simulink model "stsmc"  (R2026a)
settings: Solver=FixedStepDiscrete  FixedStep=0.001
undefined symbols (not defined in the file): DiscIntNeverNeededParam
libraries: discretizing x2
settings Model: SILPILModeSetting=veronly  Creator=HomePC  LastModifiedBy=HomePC
settings RTWCC: SystemTargetFile=ert.tlc  GenCodeOnly=on  TemplateMakefile=RTW.MSVCBuild  Toolchain=ESP32  BuildConfiguration=Faster Runs  Description=Create Visual C/C++ Solution File for Embedded Coder
settings ERTTargetCC: DynamicArrayContainerType=coder::array  GenerateSampleERTMain=on  SupportComplex=off

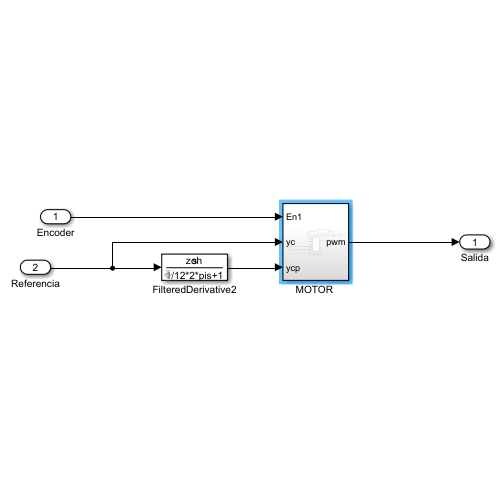
[thumbnail: Simulink's stored preview of the top-level diagram]
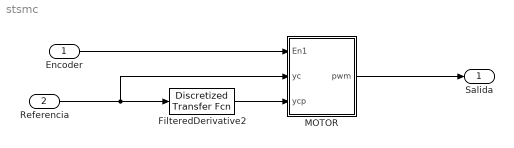
== system stsmc ==
  Encoder : Inport
  Referencia : Inport  Port=2
  FilteredDerivative2 : discretizing/Discretized Transfer Fcn  Numerator=[1 0]  Denominator=[1/12*2*pi 1]  AbsTol=auto  SampleTime=0.001  method=zoh  Wc=0
  "MOTOR " : Subsystem
  Salida : Outport
  wires:
  Encoder/1 -> "MOTOR "/1(En1)
  FilteredDerivative2/1 -> "MOTOR "/3(ycp)
  Referencia/1 -> "MOTOR "/2(yc), FilteredDerivative2/1
  "MOTOR "/1(pwm) -> Salida/1

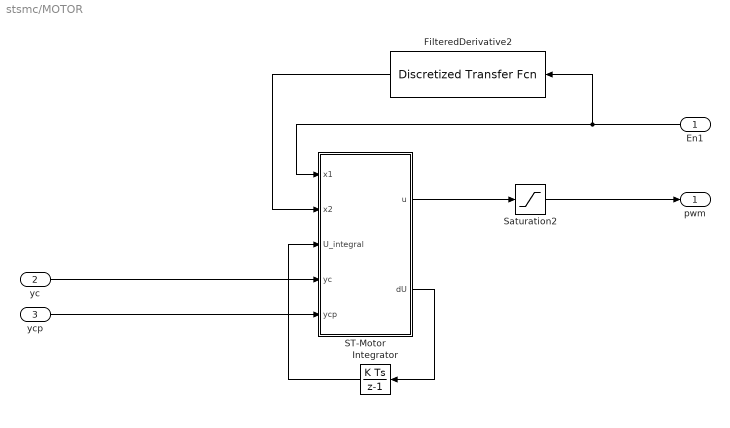
== system stsmc/MOTOR  ==
  En1 : Inport
  yc : Inport  Port=2
  ycp : Inport  Port=3
  FilteredDerivative2 : discretizing/Discretized Transfer Fcn  Numerator=[1 0]  Denominator=[1/10*2*pi 1]  AbsTol=auto  SampleTime=0.001  method=zoh  Wc=0
  Integrator : DiscreteIntegrator  gainval=1  SampleTime=0.001  ICPrevOutput=DiscIntNeverNeededParam  ICPrevScaledInput=DiscIntNeverNeededParam  mask(DiscretizedDiscreteIntegrator){}
      mask init:
      | %zoh
  ST-Motor : MATLAB Function  TreatAsAtomicUnit=on
  Saturation2 : Saturate  UpperLimit=4095  LowerLimit=-4095
  pwm : Outport  VectorParamsAs1DForOutWhenUnconnected=off
  wires:
  yc/1 -> ST-Motor/4(yc)
  ycp/1 -> ST-Motor/5(ycp)
  Integrator/1 -> ST-Motor/3(U_integral)
  ST-Motor/2(dU) -> Integrator/1
  FilteredDerivative2/1 -> ST-Motor/2(x2)
  En1/1 -> FilteredDerivative2/1, ST-Motor/1(x1)
  ST-Motor/1(u) -> Saturation2/1
  Saturation2/1 -> pwm/1

== matlab function stsmc/MOTOR /ST-Motor ==
  data: x1 input; x2 input; u output; U_integral input; yc input; ycp input; dU output
function [u, dU] = fcn(x1, x2, U_integral, yc, ycp)

    % --- 1. Sintonización (Ajustar experimentalmente) ---
    % lambda: Pendiente de la superficie. Define qué tan rápido converge el error a cero.
    lamda = 12; 
    
    % Ganancias del Super-Twisting (Regla general: k1 = 1.5*sqrt(k2))
    % Reduce alfa1 drásticamente comparado con tu versión original.
    alfa2 = 100;         % Ganancia Integral (k2). Aumenta la robustez.
    alfa1 = 15;          % Ganancia "Proporcional" (k1). 1.5 * sqrt(100) = 15
    
    % --- 2. Cálculo del Error ---
    e = yc - x1;         % OJO: Referencia - Real (Feedback Negativo)
    de = ycp - x2;       % Derivada Referencia - Derivada Real
    
    % Superficie de deslizamiento (s)
    slide = de + lamda * e;
    
    % --- 3. Algoritmo Super-Twisting ---
    % u = u_sta_1 + u_sta_2
    
    % Término 1: Raíz cuadrada (Aporta gran ganancia cerca de s=0)
    % Usamos -alfa1 para asegurar convergencia
    u_sta_proportional = alfa1 * sqrt(abs(slide)) * sign(slide);
    
    % Término 2: Integral (Derivada del término integral)
    % Esta dU debe ir a un bloque INTEGRATOR fuera de esta función
    dU = alfa2 * sign(slide); 
    
    % --- 4. Ley de Control Total ---
    % u = Integrador + Término_Raiz
    % NOTA: U_integral ya debe venir acumulado desde el paso anterior
    u = U_integral + u_sta_proportional;  

end
